simulink model "circuitomotor_simulink"  (R2026a)
settings: Solver=VariableStepAuto
InitFcn:
  | Ra=2;
  | Kt=0.01;
  | b =0.0012;
  | La=0.023;
  | Ke=0.01;
  | Jm=0.001;
  | Va=5;
settings Model: Creator=elmik  LastModifiedBy=elmik

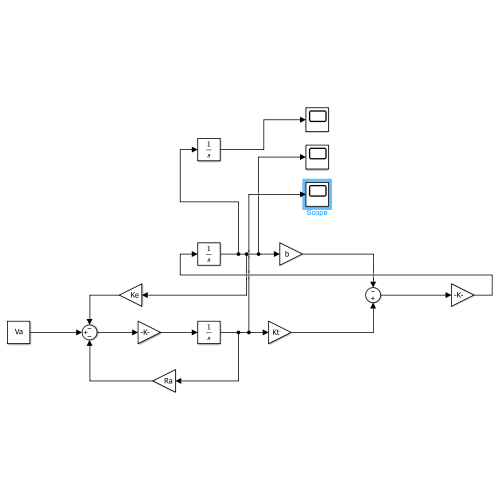
[thumbnail: Simulink's stored preview of the top-level diagram]
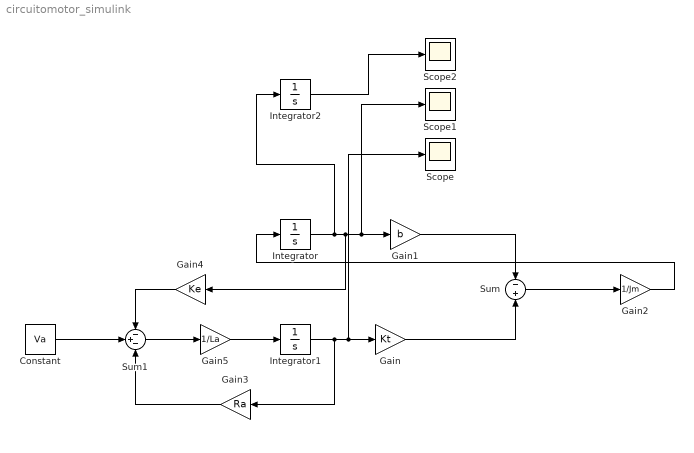
== system circuitomotor_simulink ==
  Constant : Constant  Value=Va
  Gain : Gain  Gain=Kt
  Gain1 : Gain  Gain=b
  Gain2 : Gain  Gain=1/Jm
  Gain3 : Gain  Gain=Ra
  Gain4 : Gain  Gain=Ke
  Gain5 : Gain  Gain=1/La
  Integrator : Integrator
  Integrator1 : Integrator
  Integrator2 : Integrator
  Scope : Scope
      settings: ActiveDisplayYMinimum=-0.31135564501240182  ActiveDisplayYMaximum=2.802200805111617
  Scope1 : Scope
      settings: ActiveDisplayYMinimum=-2.5000246764832204  ActiveDisplayYMaximum=22.500222088348988
  Scope2 : Scope
      settings: ActiveDisplayYMinimum=-22.972407465494872  ActiveDisplayYMaximum=206.75166718945388  DataLoggingVariableName=ScopeData2
  Sum : Sum  Inputs=-+
  Sum1 : Sum  Inputs=-+-
  wires:
  Integrator/1 -> Gain4/1, Scope1/1, Gain1/1, Integrator2/1
  Gain1/1 -> Sum/1
  Gain/1 -> Sum/2
  Sum/1 -> Gain2/1
  Gain2/1 -> Integrator/1
  Constant/1 -> Sum1/2
  Integrator1/1 -> Scope/1, Gain/1, Gain3/1
  Gain3/1 -> Sum1/3
  Gain4/1 -> Sum1/1
  Sum1/1 -> Gain5/1
  Gain5/1 -> Integrator1/1
  Integrator2/1 -> Scope2/1
